simulink model "CLVF"  (R2020a)
settings: Solver=FixedStepAuto  StartTime=0.0  StopTime=tsim  FixedStep=baseRate  RelTol=1e-3  EnableMultiTasking=on
values from neighbouring files (symbols this model uses):
  a = sqrt(sum(aTimesOVec.^2))    [Run_Initializer.m]    (also in a_max_CLVF2D.m = params(4))
  a_max = 0.4/BLACKMass    [Run_Initializer.m]
  a_prime = newParams(2)    [Run_Initializer.m]    (also in a_max_LVF.m = params(2))
  acceptableRadius = 0.05    [Run_Initializer.m]
  b = newParams(3)    [Run_Initializer.m]    (also in a_max_CLVF2D.m = params(3))
  baseRate = 0.05    [Run_Initializer.m]
  BLACKMass = model_param(3)    [Run_Initializer.m]
  d = [0.16;0.542;0]    [Run_Initializer.m]    (also in a_max_LVF.m = [rotStuff(3);rotStuff(4);rotStuff(5)])
  drop_states_BLACK = rC_I0    [Run_Initializer.m]
  drop_states_BLUE = [ xLength/2+0.9; yLength/2+0.5; 0]    [Run_Initializer.m]
  drop_states_RED = rT_I0    [Run_Initializer.m]
  F_thrusters_BLACK = 0.25.*ones(8,1)    [Run_Initializer.m]
  F_thrusters_BLUE = 0.25.*ones(8,1)    [Run_Initializer.m]
  F_thrusters_RED = 0.25.*ones(8,1)    [Run_Initializer.m]
  home_states_BLACK = [ xLength/2+0.4; yLength/2; 0]    [Run_Initializer.m]
  home_states_BLUE = [ xLength/2-0.9; yLength/2+0.5; 0]    [Run_Initializer.m]
  home_states_RED = [ xLength/2-0.4; yLength/2; 0]    [Run_Initializer.m]
  init_states_BLACK = rC_I0    [Run_Initializer.m]
  init_states_BLUE = [ xLength/2+0.9; yLength/2+0.5; 0]    [Run_Initializer.m]
  init_states_RED = rT_I0    [Run_Initializer.m]
  k_v_rel = 2*v_max/a_prime    (= 1)    [Run_Initializer.m]
  ka = newParams(2)    [Run_Initializer.m]    (also in a_max_CLVF2D.m = params(2))
  kc = newParams(1)    [Run_Initializer.m]    (also in a_max_CLVF2D.m = params(1))
  kd = 5.0    (= 5)    [Run_Initializer.m]
  Kd_tb = 0.4    [Run_Initializer.m]
  Kd_tblue = 0.4    [Run_Initializer.m]
  Kd_tr = 0.4    [Run_Initializer.m]
  Kd_xb = 5    [Run_Initializer.m]
  Kd_xblue = 5    [Run_Initializer.m]
  Kd_xr = 5    [Run_Initializer.m]
  Kd_yb = 5    [Run_Initializer.m]
  Kd_yblue = 5    [Run_Initializer.m]
  Kd_yr = 5    [Run_Initializer.m]
  Kp_tb = 0.1    [Run_Initializer.m]
  Kp_tblue = 0.1    [Run_Initializer.m]
  Kp_tr = 0.1    [Run_Initializer.m]
  Kp_xb = 2    [Run_Initializer.m]
  Kp_xblue = 2    [Run_Initializer.m]
  Kp_xr = 2    [Run_Initializer.m]
  Kp_yb = 2    [Run_Initializer.m]
  Kp_yblue = 2    [Run_Initializer.m]
  Kp_yr = 2    [Run_Initializer.m]
  noise_variance_BLACK = 0    [Run_Initializer.m]
  noise_variance_BLUE = 0    [Run_Initializer.m]
  noise_variance_RED = 0    [Run_Initializer.m]
  o_hat_B = aTimesOVec./a    [Run_Initializer.m]
  o_hat_prime = o_prime/sqrt(sum(o_prime.^2))    [Run_Initializer.m]
  Phase0_End = Phase0_Duration    (= 10)    [Run_Initializer.m]
  Phase1_End = Phase0_Duration + Phase1_Duration    (= 15)    [Run_Initializer.m]
  Phase2_End = Phase0_Duration + Phase1_Duration +                                   Phase2_Duration    (= 35)    [Run_Initializer.m]
  Phase3_End = Phase0_Duration + Phase1_Duration +                                   Phase2_Duration + Phase3_Duration    [Run_Initializer.m]
  Phase3_SubPhase1_End = Phase2_End + Phase3_SubPhase1_Duration    (= 40)    [Run_Initializer.m]
  Phase3_SubPhase2_End = Phase2_End + Phase3_SubPhase1_Duration +                                   Phase3_SubPhase2_Duration    (= 45)    [Run_Initializer.m]
  Phase3_SubPhase3_End_BLACK = Phase2_End + Phase3_SubPhase1_Duration +                                   Phase3_SubPhase2_Duration +                                  Phase3_SubPhase3_Duration + Phase3_SubPhase3_and_a_half    (= 51)    [Run_Initializer.m]
  Phase3_SubPhase3_End_RED = Phase2_End + Phase3_SubPhase1_Duration +                                   Phase3_SubPhase2_Duration +                                  Phase3_SubPhase3_Duration    (= 46)    [Run_Initializer.m]
  Phase3_SubPhase4_End = Phase2_End + Phase3_SubPhase1_Duration +                                   Phase3_SubPhase2_Duration +                                  Phase3_SubPhase3_Duration +                                  Phase3_SubPhase4_Duration + Phase3_SubPhase3_and_a_half    [Run_Initializer.m]
  Phase4_End = Phase0_Duration + Phase1_Duration +                                   Phase2_Duration + Phase3_Duration +                                   Phase4_Duration    [Run_Initializer.m]
  Phase5_End = Phase0_Duration + Phase1_Duration +                                   Phase2_Duration + Phase3_Duration +                                   Phase4_Duration + Phase5_Duration    [Run_Initializer.m]
  r_co = r_co_over_a_prime*a_prime    (= 0.16)    [Run_Initializer.m]
  rC_I0 = [0.9*xLength;yLength/2-0.5;pi/2]    [Run_Initializer.m]
  rT_I0 = [yLength/2;yLength/2;possibleStarts(startingRotation)]    [Run_Initializer.m]
  serverRate = 0.1    [Run_Initializer.m]
  sys_BLACK = c2d(sys_BLACK_CONT, baseRate)    [Run_Initializer.m]
  sys_BLACK_ROT = c2d(sys_BLACK_rot_CONT, baseRate)    [Run_Initializer.m]
  sys_RED = c2d(sys_RED_CONT, baseRate)    [Run_Initializer.m]
  sys_RED_ROT = c2d(sys_RED_rot_CONT, baseRate)    [Run_Initializer.m]
  theta_d = 30*d2r    (= 0.523598775598)    [Run_Initializer.m]    (also in a_max_LVF.m = rotStuff(2))
  thruster_dist2CG_BLACK = [83.42;-52.58;55.94;-60.05;54.08;-53.92;77.06;-55.94]    [Run_Initializer.m]
  thruster_dist2CG_BLUE = [83.42;-52.58;55.94;-60.05;54.08;-53.92;77.06;-55.94]    [Run_Initializer.m]
  thruster_dist2CG_RED = [49.92;-78.08;70.46;-63.54;81.08;-50.42;57.44;-75.96]    [Run_Initializer.m]
  w_body = 6.0 * d2r    (= 0.10471975512)    [Run_Initializer.m]
undefined symbols (not defined in the file or in its folder): DiscIntNeverNeededParam, Discrete, Phase3_SubPhase3_End, platformSelection, simMode, Time, WhoAmI
libraries: dspstat3 x18, dspsigops x14, raspberrypiBasiclib x10, embdlinuxlib x8, simulink x8, ctrlSharedLib x4, mspfiltlib x3, dsparch4 x3, dspswit3 x2, MainLibrary x2, sensehatlib x1
(part 5 of 10)

== system CLVF/Phase #4: Return Home/Change BLUE Behavior/Custom Discrete PD (Y-Position) ==
  ey : Inport
  Sum3 : Sum
  kd_yb : Gain  Gain=Kd_yblue
  kp_yb : Gain  Gain=Kp_yblue
  "x_dot -> x1" : Subsystem
  Fy : Outport  VectorParamsAs1DForOutWhenUnconnected=off
  wires:
  kd_yb/1 -> Sum3/1
  Sum3/1 -> Fy/1
  kp_yb/1 -> Sum3/2
  "x_dot -> x1"/1(dy(t)/dt) -> kd_yb/1
  ey/1 -> "x_dot -> x1"/1(y(t)), kp_yb/1

== system CLVF/Phase #4: Return Home/Change BLUE Behavior/Hough Control ==
  Ref : Inport
  Act : Inport  Port=2
  MATLAB Function2 : MATLAB Function  TreatAsAtomicUnit=on
  MATLAB Function3 : MATLAB Function  TreatAsAtomicUnit=on
  MATLAB Function4 : MATLAB Function  TreatAsAtomicUnit=on
  Subtract2 : Sum  Inputs=+-
  Err : Outport  VectorParamsAs1DForOutWhenUnconnected=off
  wires:
  MATLAB Function4/1(e_out) -> Err/1
  MATLAB Function2/1(Oy) -> MATLAB Function4/1(Oy)
  Subtract2/1 -> MATLAB Function4/2(e_in)
  MATLAB Function2/2(Ox) -> Subtract2/1
  Act/1 -> MATLAB Function3/1(z)
  Ref/1 -> MATLAB Function2/1(z)
  MATLAB Function3/1(Ox) -> Subtract2/2

== system CLVF/Phase #4: Return Home/Change RED Behavior/Custom Discrete PD (Attitude) ==
  ez : Inport
  Sum3 : Sum
  kd_tr : Gain  Gain=Kd_tr
  kp_tr : Gain  Gain=Kp_tr
  "x_dot -> x1" : Subsystem
  Tz : Outport  VectorParamsAs1DForOutWhenUnconnected=off
  wires:
  kd_tr/1 -> Sum3/1
  Sum3/1 -> Tz/1
  kp_tr/1 -> Sum3/2
  "x_dot -> x1"/1(dy(t)/dt) -> kd_tr/1
  ez/1 -> "x_dot -> x1"/1(y(t)), kp_tr/1

== system CLVF/Phase #4: Return Home/Change RED Behavior/Custom Discrete PD (X-Position) ==
  ex : Inport
  Sum3 : Sum
  kd_xr : Gain  Gain=Kd_xr
  kp_xr : Gain  Gain=Kp_xr
  "x_dot -> x1" : Subsystem
  Fx : Outport  VectorParamsAs1DForOutWhenUnconnected=off
  wires:
  kd_xr/1 -> Sum3/1
  ex/1 -> "x_dot -> x1"/1(y(t)), kp_xr/1
  kp_xr/1 -> Sum3/2
  "x_dot -> x1"/1(dy(t)/dt) -> kd_xr/1
  Sum3/1 -> Fx/1

== system CLVF/Phase #4: Return Home/Change RED Behavior/Custom Discrete PD (Y-Position) ==
  ey : Inport
  Sum3 : Sum
  kd_yr : Gain  Gain=Kd_yr
  kp_yr : Gain  Gain=Kp_yr
  "x_dot -> x1" : Subsystem
  Fy : Outport  VectorParamsAs1DForOutWhenUnconnected=off
  wires:
  kd_yr/1 -> Sum3/1
  Sum3/1 -> Fy/1
  kp_yr/1 -> Sum3/2
  "x_dot -> x1"/1(dy(t)/dt) -> kd_yr/1
  ey/1 -> "x_dot -> x1"/1(y(t)), kp_yr/1

== system CLVF/Phase #4: Return Home/Change RED Behavior/Hough Control ==
  Ref : Inport
  Act : Inport  Port=2
  MATLAB Function2 : MATLAB Function  TreatAsAtomicUnit=on
  MATLAB Function3 : MATLAB Function  TreatAsAtomicUnit=on
  MATLAB Function4 : MATLAB Function  TreatAsAtomicUnit=on
  Subtract2 : Sum  Inputs=+-
  Err : Outport  VectorParamsAs1DForOutWhenUnconnected=off
  wires:
  MATLAB Function4/1(e_out) -> Err/1
  MATLAB Function2/1(Oy) -> MATLAB Function4/1(Oy)
  Subtract2/1 -> MATLAB Function4/2(e_in)
  MATLAB Function2/2(Ox) -> Subtract2/1
  Act/1 -> MATLAB Function3/1(z)
  Ref/1 -> MATLAB Function2/1(z)
  MATLAB Function3/1(Ox) -> Subtract2/2

== system CLVF/Phase #5: Hold Home/Change BLACK Behavior/Custom Discrete PD (Attitude) ==
  ez : Inport
  Sum3 : Sum
  kd_tb : Gain  Gain=Kd_tb
  kp_tb : Gain  Gain=Kp_tb
  "x_dot -> x1" : Subsystem
  Tz : Outport  VectorParamsAs1DForOutWhenUnconnected=off
  wires:
  kd_tb/1 -> Sum3/1
  Sum3/1 -> Tz/1
  kp_tb/1 -> Sum3/2
  "x_dot -> x1"/1(dy(t)/dt) -> kd_tb/1
  ez/1 -> "x_dot -> x1"/1(y(t)), kp_tb/1

== system CLVF/Phase #5: Hold Home/Change BLACK Behavior/Custom Discrete PD (X-Position) ==
  ex : Inport
  Sum3 : Sum
  kd_xb : Gain  Gain=Kd_xb
  kp_xb : Gain  Gain=Kp_xb
  "x_dot -> x1" : Subsystem
  Fx : Outport  VectorParamsAs1DForOutWhenUnconnected=off
  wires:
  kd_xb/1 -> Sum3/1
  ex/1 -> "x_dot -> x1"/1(y(t)), kp_xb/1
  kp_xb/1 -> Sum3/2
  "x_dot -> x1"/1(dy(t)/dt) -> kd_xb/1
  Sum3/1 -> Fx/1

== system CLVF/Phase #5: Hold Home/Change BLACK Behavior/Custom Discrete PD (Y-Position) ==
  ey : Inport
  Sum3 : Sum
  kd_yb : Gain  Gain=Kd_yb
  kp_yb : Gain  Gain=Kp_yb
  "x_dot -> x1" : Subsystem
  Fy : Outport  VectorParamsAs1DForOutWhenUnconnected=off
  wires:
  kd_yb/1 -> Sum3/1
  Sum3/1 -> Fy/1
  kp_yb/1 -> Sum3/2
  "x_dot -> x1"/1(dy(t)/dt) -> kd_yb/1
  ey/1 -> "x_dot -> x1"/1(y(t)), kp_yb/1

== system CLVF/Phase #5: Hold Home/Change BLACK Behavior/Hough Control ==
  Ref : Inport
  Act : Inport  Port=2
  MATLAB Function2 : MATLAB Function  TreatAsAtomicUnit=on
  MATLAB Function3 : MATLAB Function  TreatAsAtomicUnit=on
  MATLAB Function4 : MATLAB Function  TreatAsAtomicUnit=on
  Subtract2 : Sum  Inputs=+-
  Err : Outport  VectorParamsAs1DForOutWhenUnconnected=off
  wires:
  MATLAB Function4/1(e_out) -> Err/1
  MATLAB Function2/1(Oy) -> MATLAB Function4/1(Oy)
  Subtract2/1 -> MATLAB Function4/2(e_in)
  MATLAB Function2/2(Ox) -> Subtract2/1
  Act/1 -> MATLAB Function3/1(z)
  Ref/1 -> MATLAB Function2/1(z)
  MATLAB Function3/1(Ox) -> Subtract2/2

== system CLVF/Phase #5: Hold Home/Change BLUE Behavior/Custom Discrete PD (Attitude) ==
  ez : Inport
  Sum3 : Sum
  kd_tb : Gain  Gain=Kd_tblue
  kp_tb : Gain  Gain=Kp_tblue
  "x_dot -> x1" : Subsystem
  Tz : Outport  VectorParamsAs1DForOutWhenUnconnected=off
  wires:
  kd_tb/1 -> Sum3/1
  Sum3/1 -> Tz/1
  kp_tb/1 -> Sum3/2
  "x_dot -> x1"/1(dy(t)/dt) -> kd_tb/1
  ez/1 -> "x_dot -> x1"/1(y(t)), kp_tb/1

== system CLVF/Phase #5: Hold Home/Change BLUE Behavior/Custom Discrete PD (X-Position) ==
  ex : Inport
  Sum3 : Sum
  kd_xb : Gain  Gain=Kd_xblue
  kp_xb : Gain  Gain=Kp_xblue
  "x_dot -> x1" : Subsystem
  Fx : Outport  VectorParamsAs1DForOutWhenUnconnected=off
  wires:
  kd_xb/1 -> Sum3/1
  ex/1 -> "x_dot -> x1"/1(y(t)), kp_xb/1
  kp_xb/1 -> Sum3/2
  "x_dot -> x1"/1(dy(t)/dt) -> kd_xb/1
  Sum3/1 -> Fx/1

== system CLVF/Phase #5: Hold Home/Change BLUE Behavior/Custom Discrete PD (Y-Position) ==
  ey : Inport
  Sum3 : Sum
  kd_yb : Gain  Gain=Kd_yblue
  kp_yb : Gain  Gain=Kp_yblue
  "x_dot -> x1" : Subsystem
  Fy : Outport  VectorParamsAs1DForOutWhenUnconnected=off
  wires:
  kd_yb/1 -> Sum3/1
  Sum3/1 -> Fy/1
  kp_yb/1 -> Sum3/2
  "x_dot -> x1"/1(dy(t)/dt) -> kd_yb/1
  ey/1 -> "x_dot -> x1"/1(y(t)), kp_yb/1

== system CLVF/Phase #5: Hold Home/Change BLUE Behavior/Hough Control ==
  Ref : Inport
  Act : Inport  Port=2
  MATLAB Function2 : MATLAB Function  TreatAsAtomicUnit=on
  MATLAB Function3 : MATLAB Function  TreatAsAtomicUnit=on
  MATLAB Function4 : MATLAB Function  TreatAsAtomicUnit=on
  Subtract2 : Sum  Inputs=+-
  Err : Outport  VectorParamsAs1DForOutWhenUnconnected=off
  wires:
  MATLAB Function4/1(e_out) -> Err/1
  MATLAB Function2/1(Oy) -> MATLAB Function4/1(Oy)
  Subtract2/1 -> MATLAB Function4/2(e_in)
  MATLAB Function2/2(Ox) -> Subtract2/1
  Act/1 -> MATLAB Function3/1(z)
  Ref/1 -> MATLAB Function2/1(z)
  MATLAB Function3/1(Ox) -> Subtract2/2

== system CLVF/Phase #5: Hold Home/Change RED Behavior/Custom Discrete PD (Attitude) ==
  ez : Inport
  Sum3 : Sum
  kd_tr : Gain  Gain=Kd_tr
  kp_tr : Gain  Gain=Kp_tr
  "x_dot -> x1" : Subsystem
  Tz : Outport  VectorParamsAs1DForOutWhenUnconnected=off
  wires:
  kd_tr/1 -> Sum3/1
  Sum3/1 -> Tz/1
  kp_tr/1 -> Sum3/2
  "x_dot -> x1"/1(dy(t)/dt) -> kd_tr/1
  ez/1 -> "x_dot -> x1"/1(y(t)), kp_tr/1

== system CLVF/Phase #5: Hold Home/Change RED Behavior/Custom Discrete PD (X-Position) ==
  ex : Inport
  Sum3 : Sum
  kd_xr : Gain  Gain=Kd_xr
  kp_xr : Gain  Gain=Kp_xr
  "x_dot -> x1" : Subsystem
  Fx : Outport  VectorParamsAs1DForOutWhenUnconnected=off
  wires:
  kd_xr/1 -> Sum3/1
  ex/1 -> "x_dot -> x1"/1(y(t)), kp_xr/1
  kp_xr/1 -> Sum3/2
  "x_dot -> x1"/1(dy(t)/dt) -> kd_xr/1
  Sum3/1 -> Fx/1

== system CLVF/Phase #5: Hold Home/Change RED Behavior/Custom Discrete PD (Y-Position) ==
  ey : Inport
  Sum3 : Sum
  kd_yr : Gain  Gain=Kd_yr
  kp_yr : Gain  Gain=Kp_yr
  "x_dot -> x1" : Subsystem
  Fy : Outport  VectorParamsAs1DForOutWhenUnconnected=off
  wires:
  kd_yr/1 -> Sum3/1
  Sum3/1 -> Fy/1
  kp_yr/1 -> Sum3/2
  "x_dot -> x1"/1(dy(t)/dt) -> kd_yr/1
  ey/1 -> "x_dot -> x1"/1(y(t)), kp_yr/1

== system CLVF/Phase #5: Hold Home/Change RED Behavior/Hough Control ==
  Ref : Inport
  Act : Inport  Port=2
  MATLAB Function2 : MATLAB Function  TreatAsAtomicUnit=on
  MATLAB Function3 : MATLAB Function  TreatAsAtomicUnit=on
  MATLAB Function4 : MATLAB Function  TreatAsAtomicUnit=on
  Subtract2 : Sum  Inputs=+-
  Err : Outport  VectorParamsAs1DForOutWhenUnconnected=off
  wires:
  MATLAB Function4/1(e_out) -> Err/1
  MATLAB Function2/1(Oy) -> MATLAB Function4/1(Oy)
  Subtract2/1 -> MATLAB Function4/2(e_in)
  MATLAB Function2/2(Ox) -> Subtract2/1
  Act/1 -> MATLAB Function3/1(z)
  Ref/1 -> MATLAB Function2/1(z)
  MATLAB Function3/1(Ox) -> Subtract2/2

== system CLVF/Simulate Plant Dynamics/x_dot -> x1/Hold this value ==
  In1 : Inport
  Action Port : ActionPort
  Out1 : Outport  VectorParamsAs1DForOutWhenUnconnected=off
  wires:
  In1/1 -> Out1/1

== system CLVF/Simulate Plant Dynamics/x_dot -> x10/Hold this value ==
  In1 : Inport
  Action Port : ActionPort
  Out1 : Outport  VectorParamsAs1DForOutWhenUnconnected=off
  wires:
  In1/1 -> Out1/1

== system CLVF/Simulate Plant Dynamics/x_dot -> x11/Hold this value ==
  In1 : Inport
  Action Port : ActionPort
  Out1 : Outport  VectorParamsAs1DForOutWhenUnconnected=off
  wires:
  In1/1 -> Out1/1

== system CLVF/Simulate Plant Dynamics/x_dot -> x13/Hold this value ==
  In1 : Inport
  Action Port : ActionPort
  Out1 : Outport  VectorParamsAs1DForOutWhenUnconnected=off
  wires:
  In1/1 -> Out1/1

== system CLVF/Simulate Plant Dynamics/x_dot -> x14/Hold this value ==
  In1 : Inport
  Action Port : ActionPort
  Out1 : Outport  VectorParamsAs1DForOutWhenUnconnected=off
  wires:
  In1/1 -> Out1/1

== system CLVF/Simulate Plant Dynamics/x_dot -> x16/Hold this value ==
  In1 : Inport
  Action Port : ActionPort
  Out1 : Outport  VectorParamsAs1DForOutWhenUnconnected=off
  wires:
  In1/1 -> Out1/1

== system CLVF/Simulate Plant Dynamics/x_dot -> x17/Hold this value ==
  In1 : Inport
  Action Port : ActionPort
  Out1 : Outport  VectorParamsAs1DForOutWhenUnconnected=off
  wires:
  In1/1 -> Out1/1

== system CLVF/Simulate Plant Dynamics/x_dot -> x2/Hold this value ==
  In1 : Inport
  Action Port : ActionPort
  Out1 : Outport  VectorParamsAs1DForOutWhenUnconnected=off
  wires:
  In1/1 -> Out1/1

== system CLVF/Simulate Plant Dynamics/x_dot -> x3/Hold this value ==
  In1 : Inport
  Action Port : ActionPort
  Out1 : Outport  VectorParamsAs1DForOutWhenUnconnected=off
  wires:
  In1/1 -> Out1/1

== system CLVF/Simulate Plant Dynamics/x_dot -> x4/Hold this value ==
  In1 : Inport
  Action Port : ActionPort
  Out1 : Outport  VectorParamsAs1DForOutWhenUnconnected=off
  wires:
  In1/1 -> Out1/1

== system CLVF/Simulate Plant Dynamics/x_dot -> x5/Hold this value ==
  In1 : Inport
  Action Port : ActionPort
  Out1 : Outport  VectorParamsAs1DForOutWhenUnconnected=off
  wires:
  In1/1 -> Out1/1

== system CLVF/Simulate Plant Dynamics/x_dot -> x6/Hold this value ==
  In1 : Inport
  Action Port : ActionPort
  Out1 : Outport  VectorParamsAs1DForOutWhenUnconnected=off
  wires:
  In1/1 -> Out1/1

== system CLVF/Simulate Plant Dynamics/x_dot -> x7/Hold this value ==
  In1 : Inport
  Action Port : ActionPort
  Out1 : Outport  VectorParamsAs1DForOutWhenUnconnected=off
  wires:
  In1/1 -> Out1/1

== system CLVF/Simulate Plant Dynamics/x_dot -> x8/Hold this value ==
  In1 : Inport
  Action Port : ActionPort
  Out1 : Outport  VectorParamsAs1DForOutWhenUnconnected=off
  wires:
  In1/1 -> Out1/1

== system CLVF/Simulate Plant Dynamics/x_dot -> x9/Hold this value ==
  In1 : Inport
  Action Port : ActionPort
  Out1 : Outport  VectorParamsAs1DForOutWhenUnconnected=off
  wires:
  In1/1 -> Out1/1

== system CLVF/From Force//Torque to PWM Signal/Change BLACK Behavior/Calculate Thruster ON//OFF/Rotate Forces to Inertial ==
  "F_b " : Inport
  Rz : Inport  Port=2
  Create Rotation Matrix : MATLAB Function  TreatAsAtomicUnit=on
  Rotate F_b to F_I : Product  Multiplication=Matrix(*)
  F_I : Outport  VectorParamsAs1DForOutWhenUnconnected=off
  wires:
  "F_b "/1 -> Rotate F_b to F_I/2
  Rotate F_b to F_I/1 -> F_I/1
  Create Rotation Matrix/1(C_Ib) -> Rotate F_b to F_I/1
  Rz/1 -> Create Rotation Matrix/1(Rz)

== system CLVF/From Force//Torque to PWM Signal/Change BLACK Behavior/Calculate Thruster ON//OFF/pseudo-inverse ==
  H : Inport
  Product : Product  Multiplication=Matrix(*)
  Product1 : Product  Inputs=/  Multiplication=Matrix(*)
  Product2 : Product  Multiplication=Matrix(*)
  transpose : PermuteDimensions
  invH : Outport  VectorParamsAs1DForOutWhenUnconnected=off
  wires:
  Product2/1 -> invH/1
  transpose/1 -> Product/2, Product2/1
  Product/1 -> Product1/1
  H/1 -> Product/1, transpose/1
  Product1/1 -> Product2/2

== system CLVF/From Force//Torque to PWM Signal/Change BLUE Behavior/Calculate Thruster ON//OFF/Rotate Forces to Inertial ==
  "F_b " : Inport
  Rz : Inport  Port=2
  Create Rotation Matrix : MATLAB Function  TreatAsAtomicUnit=on
  Rotate F_b to F_I : Product  Multiplication=Matrix(*)
  F_I : Outport  VectorParamsAs1DForOutWhenUnconnected=off
  wires:
  "F_b "/1 -> Rotate F_b to F_I/2
  Rotate F_b to F_I/1 -> F_I/1
  Create Rotation Matrix/1(C_Ib) -> Rotate F_b to F_I/1
  Rz/1 -> Create Rotation Matrix/1(Rz)

== system CLVF/From Force//Torque to PWM Signal/Change BLUE Behavior/Calculate Thruster ON//OFF/pseudo-inverse ==
  H : Inport
  Product : Product  Multiplication=Matrix(*)
  Product1 : Product  Inputs=/  Multiplication=Matrix(*)
  Product2 : Product  Multiplication=Matrix(*)
  transpose : PermuteDimensions
  invH : Outport  VectorParamsAs1DForOutWhenUnconnected=off
  wires:
  Product2/1 -> invH/1
  transpose/1 -> Product/2, Product2/1
  Product/1 -> Product1/1
  H/1 -> Product/1, transpose/1
  Product1/1 -> Product2/2

== system CLVF/From Force//Torque to PWM Signal/Change RED Behavior/Calculate Thruster ON//OFF/Rotate Forces to Inertial ==
  "F_b " : Inport
  Rz : Inport  Port=2
  Create Rotation Matrix : MATLAB Function  TreatAsAtomicUnit=on
  Rotate F_b to F_I : Product  Multiplication=Matrix(*)
  F_I : Outport  VectorParamsAs1DForOutWhenUnconnected=off
  wires:
  "F_b "/1 -> Rotate F_b to F_I/2
  Rotate F_b to F_I/1 -> F_I/1
  Create Rotation Matrix/1(C_Ib) -> Rotate F_b to F_I/1
  Rz/1 -> Create Rotation Matrix/1(Rz)

== system CLVF/From Force//Torque to PWM Signal/Change RED Behavior/Calculate Thruster ON//OFF/pseudo-inverse ==
  H : Inport
  Product : Product  Multiplication=Matrix(*)
  Product1 : Product  Inputs=/  Multiplication=Matrix(*)
  Product2 : Product  Multiplication=Matrix(*)
  transpose : PermuteDimensions
  invH : Outport  VectorParamsAs1DForOutWhenUnconnected=off
  wires:
  Product2/1 -> invH/1
  transpose/1 -> Product/2, Product2/1
  Product/1 -> Product1/1
  H/1 -> Product/1, transpose/1
  Product1/1 -> Product2/2

== system CLVF/From Torque, Command RW/Change RED Behavior/Wheel RPM to PWM/Convert Wheel Rate to Motor Rate ==
  Wheel RPM : Inport
  Divide : Product  Inputs=**
  Gearbox Ratio : Constant  Value=3375/64
  Motor RPM : Outport  VectorParamsAs1DForOutWhenUnconnected=off
  wires:
  Gearbox Ratio/1 -> Divide/2
  Divide/1 -> Motor RPM/1
  Wheel RPM/1 -> Divide/1

== system CLVF/From Torque, Command RW/Change RED Behavior/Wheel RPM to PWM/Delay Bank ==
  Status : Inport
  Delay1 : Delay  DelayLength=1  InitialCondition=0
  Delay2 : Delay  InitialCondition=0
  Delay3 : Delay  DelayLength=4  InitialCondition=0
  Delay4 : Delay  DelayLength=5  InitialCondition=0
  Delay5 : Delay  DelayLength=3  InitialCondition=0
  Mostly zeros? : MinMax  Inputs=6
  StatusVector : Outport  VectorParamsAs1DForOutWhenUnconnected=off
  wires:
  Delay3/1 -> Mostly zeros?/5
  Status/1 -> Delay4/1, Delay3/1, Delay5/1, Delay2/1, Delay1/1, Mostly zeros?/1
  Delay2/1 -> Mostly zeros?/3
  Delay4/1 -> Mostly zeros?/6
  Delay5/1 -> Mostly zeros?/4
  Mostly zeros?/1 -> StatusVector/1
  Delay1/1 -> Mostly zeros?/2

== system CLVF/From Torque, Command RW/Change RED Behavior/Wheel RPM to PWM/Obtain RW Status ==
  GPIO Read1 : embdlinuxlib/GPIO Read  board=Pi 3 Model B  gpio=24  internalResistor=Off  sampleTime=0.1  direction=Input  blockPlatform=Raspberry Pi
      settings: SourceProductBaseCode=SC_BEAGLEBONE_BLUE,RASPPI
  RW_Status : Outport  VectorParamsAs1DForOutWhenUnconnected=off
  wires:
  GPIO Read1/1 -> RW_Status/1

== system CLVF/From Torque, Command RW/Change RED Behavior/Wheel RPM to PWM/Send Direction to Motor Controller ==
  WheelDir : Inport
  GPIO Write : embdlinuxlib/GPIO Write  board=Pi 3 Model B  gpio=21  direction=Output  blockPlatform=Raspberry Pi
      settings: SourceProductBaseCode=SC_BEAGLEBONE_BLUE,RASPPI
  wires:
  WheelDir/1 -> GPIO Write/1

== system CLVF/From Torque, Command RW/Change RED Behavior/Wheel RPM to PWM/Send PWM to Motor Controller ==
  MotorPWM : Inport
  PWM1 : raspberrypiBasiclib/PWM  board=Pi 3 Model B  Pin_=18  Frequency=10  blockPlatform=Raspberry Pi
      settings: SourceProductBaseCode=RASPPI
  wires:
  MotorPWM/1 -> PWM1/1

== system CLVF/From Torque, Command RW/Change RED Behavior/Wheel RPM to PWM/Turn on Motor ==
  EnableSig : Inport
  GPIO Write1 : embdlinuxlib/GPIO Write  board=Pi 3 Model B  gpio=25  direction=Output  blockPlatform=Raspberry Pi
      settings: SourceProductBaseCode=SC_BEAGLEBONE_BLUE,RASPPI
  wires:
  EnableSig/1 -> GPIO Write1/1

== system CLVF/Grab PhaseSpace Data via UDP/Use Hardware to Obtain States/Using RED+BLACK, or RED+BLACK+ARM/Is this a simulation? ==
  Constant : Constant  Value=simMode  SampleTime=-1
  isSim : Outport  VectorParamsAs1DForOutWhenUnconnected=off
  wires:
  Constant/1 -> isSim/1

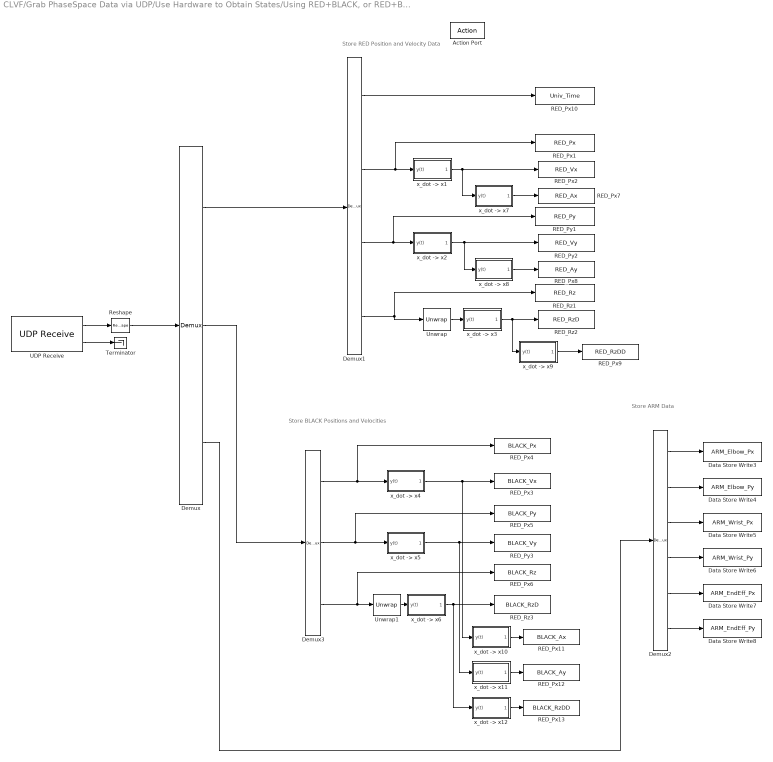
== system CLVF/Grab PhaseSpace Data via UDP/Use Hardware to Obtain States/Using RED+BLACK, or RED+BLACK+ARM/Obtain BLACK States ==
  note: Store ARM Data
  note: Store RED Position and Velocity Data
  note: Store BLACK Positions and Velocities
  Action Port : ActionPort
  Data Store Write3 : DataStoreWrite  DataStoreName=ARM_Elbow_Px
  Data Store Write4 : DataStoreWrite  DataStoreName=ARM_Elbow_Py
  Data Store Write5 : DataStoreWrite  DataStoreName=ARM_Wrist_Px
  Data Store Write6 : DataStoreWrite  DataStoreName=ARM_Wrist_Py
  Data Store Write7 : DataStoreWrite  DataStoreName=ARM_EndEff_Px
  Data Store Write8 : DataStoreWrite  DataStoreName=ARM_EndEff_Py
  Demux : Demux  Outputs=[4,3,6]
  Demux1 : Demux
  Demux2 : Demux  Outputs=6
  Demux3 : Demux  Outputs=3
  RED_Px1 : DataStoreWrite  DataStoreName=RED_Px
  RED_Px10 : DataStoreWrite  DataStoreName=Univ_Time
  RED_Px11 : DataStoreWrite  DataStoreName=BLACK_Ax
  RED_Px12 : DataStoreWrite  DataStoreName=BLACK_Ay
  RED_Px13 : DataStoreWrite  DataStoreName=BLACK_RzDD
  RED_Px2 : DataStoreWrite  DataStoreName=RED_Vx
  RED_Px3 : DataStoreWrite  DataStoreName=BLACK_Vx
  RED_Px4 : DataStoreWrite  DataStoreName=BLACK_Px
  RED_Px5 : DataStoreWrite  DataStoreName=BLACK_Py
  RED_Px6 : DataStoreWrite  DataStoreName=BLACK_Rz
  RED_Px7 : DataStoreWrite  DataStoreName=RED_Ax
  RED_Px8 : DataStoreWrite  DataStoreName=RED_Ay
  RED_Px9 : DataStoreWrite  DataStoreName=RED_RzDD
  RED_Py1 : DataStoreWrite  DataStoreName=RED_Py
  RED_Py2 : DataStoreWrite  DataStoreName=RED_Vy
  RED_Py3 : DataStoreWrite  DataStoreName=BLACK_Vy
  RED_Rz1 : DataStoreWrite  DataStoreName=RED_Rz
  RED_Rz2 : DataStoreWrite  DataStoreName=RED_RzD
  RED_Rz3 : DataStoreWrite  DataStoreName=BLACK_RzD
  Reshape : Reshape  OutputDimensionality=Customize  OutputDimensions=[13,1]
  Terminator : Terminator
  UDP Receive : embdlinuxlib/UDP Receive  localURL='0.0.0.0'  localPort=25000  remoteURL='0.0.0.0'  remotePort=-1  recvBufferSize=8192  signalDatatype=double  dims=13  isVarSize=off  showBlockingTime=off  blockingTime=0  sampletime=-1  blockPlatform=Raspberry Pi
      settings: SourceProductBaseCode=SC_BEAGLEBONE_BLUE,RASPPI
  Unwrap : dspsigops/Unwrap  tol=pi  InputProcessing=Columns as channels (frame based)  running=off
  Unwrap1 : dspsigops/Unwrap  tol=pi  InputProcessing=Columns as channels (frame based)  running=off
  "x_dot -> x1" : Subsystem
  "x_dot -> x10" : Subsystem
  "x_dot -> x11" : Subsystem
  "x_dot -> x12" : Subsystem
  "x_dot -> x2" : Subsystem
  "x_dot -> x3" : Subsystem
  "x_dot -> x4" : Subsystem
  "x_dot -> x5" : Subsystem
  "x_dot -> x6" : Subsystem
  "x_dot -> x7" : Subsystem
  "x_dot -> x8" : Subsystem
  "x_dot -> x9" : Subsystem
  wires:
  UDP Receive/1 -> Reshape/1
  UDP Receive/2 -> Terminator/1
  "x_dot -> x8"/1(dy(t)/dt) -> RED_Px8/1
  Demux2/2 -> Data Store Write4/1
  Reshape/1 -> Demux/1
  Demux1/4 -> Unwrap/1, RED_Rz1/1
  Demux1/1 -> RED_Px10/1
  Unwrap/1 -> "x_dot -> x3"/1(y(t))
  "x_dot -> x7"/1(dy(t)/dt) -> RED_Px7/1
  Demux/2 -> Demux3/1
  "x_dot -> x9"/1(dy(t)/dt) -> RED_Px9/1
  Demux/1 -> Demux1/1
  Demux/3 -> Demux2/1
  "x_dot -> x3"/1(dy(t)/dt) -> "x_dot -> x9"/1(y(t)), RED_Rz2/1
  "x_dot -> x1"/1(dy(t)/dt) -> "x_dot -> x7"/1(y(t)), RED_Px2/1
  Demux1/2 -> "x_dot -> x1"/1(y(t)), RED_Px1/1
  Demux2/4 -> Data Store Write6/1
  Demux2/6 -> Data Store Write8/1
  "x_dot -> x2"/1(dy(t)/dt) -> "x_dot -> x8"/1(y(t)), RED_Py2/1
  Demux2/3 -> Data Store Write5/1
  Demux1/3 -> "x_dot -> x2"/1(y(t)), RED_Py1/1
  Demux2/1 -> Data Store Write3/1
  Demux2/5 -> Data Store Write7/1
  "x_dot -> x11"/1(dy(t)/dt) -> RED_Px12/1
  Demux3/2 -> "x_dot -> x5"/1(y(t)), RED_Px5/1
  Demux3/3 -> Unwrap1/1, RED_Px6/1
  "x_dot -> x5"/1(dy(t)/dt) -> RED_Py3/1, "x_dot -> x11"/1(y(t))
  "x_dot -> x4"/1(dy(t)/dt) -> "x_dot -> x10"/1(y(t)), RED_Px3/1
  "x_dot -> x6"/1(dy(t)/dt) -> RED_Rz3/1, "x_dot -> x12"/1(y(t))
  Unwrap1/1 -> "x_dot -> x6"/1(y(t))
  "x_dot -> x12"/1(dy(t)/dt) -> RED_Px13/1
  Demux3/1 -> "x_dot -> x4"/1(y(t)), RED_Px4/1
  "x_dot -> x10"/1(dy(t)/dt) -> RED_Px11/1

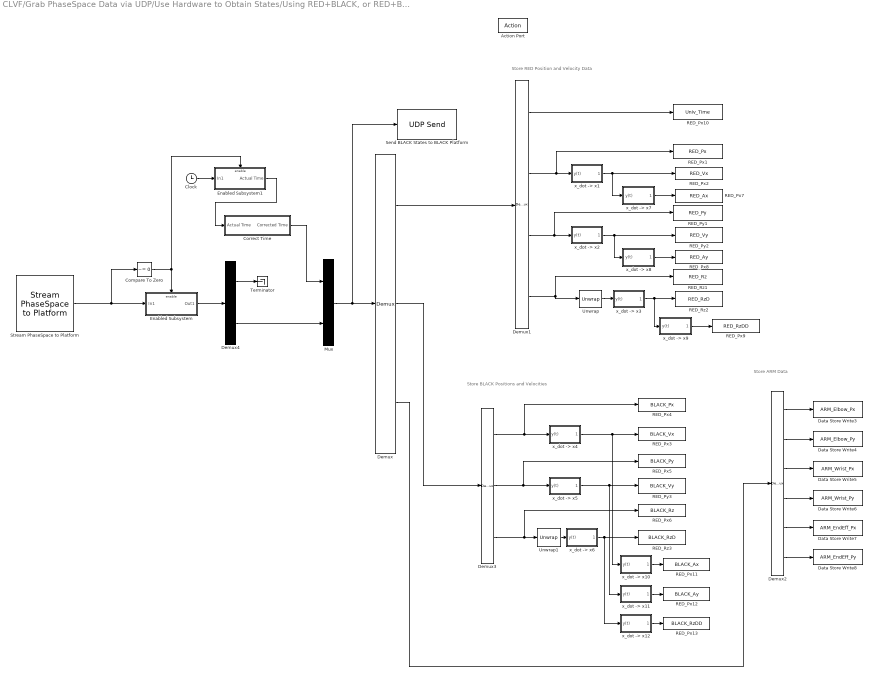
== system CLVF/Grab PhaseSpace Data via UDP/Use Hardware to Obtain States/Using RED+BLACK, or RED+BLACK+ARM/Obtain RED States ==
  note: Store ARM Data
  note: Store RED Position and Velocity Data
  note: Store BLACK Positions and Velocities
  Action Port : ActionPort
  Clock : Clock
  Compare To Zero : simulink/Logic and Bit Operations/Compare To Zero  relop=~=  OutDataTypeStr=boolean
  Correct Time : Subsystem
  Data Store Write3 : DataStoreWrite  DataStoreName=ARM_Elbow_Px
  Data Store Write4 : DataStoreWrite  DataStoreName=ARM_Elbow_Py
  Data Store Write5 : DataStoreWrite  DataStoreName=ARM_Wrist_Px
  Data Store Write6 : DataStoreWrite  DataStoreName=ARM_Wrist_Py
  Data Store Write7 : DataStoreWrite  DataStoreName=ARM_EndEff_Px
  Data Store Write8 : DataStoreWrite  DataStoreName=ARM_EndEff_Py
  Demux : Demux  Outputs=[4,3,6]
  Demux1 : Demux
  Demux2 : Demux  Outputs=6
  Demux3 : Demux  Outputs=3
  Demux4 : Demux  Outputs=[1,12]
  Enabled Subsystem : Subsystem  TreatAsAtomicUnit=on
  Enabled Subsystem1 : Subsystem  TreatAsAtomicUnit=on
  Mux : Mux  Inputs=2
  RED_Px1 : DataStoreWrite  DataStoreName=RED_Px
  RED_Px10 : DataStoreWrite  DataStoreName=Univ_Time
  RED_Px11 : DataStoreWrite  DataStoreName=BLACK_Ax
  RED_Px12 : DataStoreWrite  DataStoreName=BLACK_Ay
  RED_Px13 : DataStoreWrite  DataStoreName=BLACK_RzDD
  RED_Px2 : DataStoreWrite  DataStoreName=RED_Vx
  RED_Px3 : DataStoreWrite  DataStoreName=BLACK_Vx
  RED_Px4 : DataStoreWrite  DataStoreName=BLACK_Px
  RED_Px5 : DataStoreWrite  DataStoreName=BLACK_Py
  RED_Px6 : DataStoreWrite  DataStoreName=BLACK_Rz
  RED_Px7 : DataStoreWrite  DataStoreName=RED_Ax
  RED_Px8 : DataStoreWrite  DataStoreName=RED_Ay
  RED_Px9 : DataStoreWrite  DataStoreName=RED_RzDD
  RED_Py1 : DataStoreWrite  DataStoreName=RED_Py
  RED_Py2 : DataStoreWrite  DataStoreName=RED_Vy
  RED_Py3 : DataStoreWrite  DataStoreName=BLACK_Vy
  RED_Rz1 : DataStoreWrite  DataStoreName=RED_Rz
  RED_Rz2 : DataStoreWrite  DataStoreName=RED_RzD
  RED_Rz3 : DataStoreWrite  DataStoreName=BLACK_RzD
  Send BLACK States to BLACK Platform : embdlinuxlib/UDP Send  remoteURL='192.168.0.101'  remotePort=25000  localURL='255.255.255.255'  localPortSource=Automatically determine  localPort=-1  sampletime=-1  blockPlatform=Raspberry Pi  separateLengthPort=0
      settings: SourceProductBaseCode=SC_BEAGLEBONE_BLUE,RASPPI
  Stream PhaseSpace to Platform : MainLibrary/PhaseSpace Functions/Stream PhaseSpace to Platform  platformSelection=platformSelection  PS_SampleRate=1/serverRate
      settings: SourceProductName=SPOT Custom Library
  Terminator : Terminator
  Unwrap : dspsigops/Unwrap  tol=pi  InputProcessing=Columns as channels (frame based)  running=off
  Unwrap1 : dspsigops/Unwrap  tol=pi  InputProcessing=Columns as channels (frame based)  running=off
  "x_dot -> x1" : Subsystem
  "x_dot -> x10" : Subsystem
  "x_dot -> x11" : Subsystem
  "x_dot -> x12" : Subsystem
  "x_dot -> x2" : Subsystem
  "x_dot -> x3" : Subsystem
  "x_dot -> x4" : Subsystem
  "x_dot -> x5" : Subsystem
  "x_dot -> x6" : Subsystem
  "x_dot -> x7" : Subsystem
  "x_dot -> x8" : Subsystem
  "x_dot -> x9" : Subsystem
  wires:
  "x_dot -> x8"/1(dy(t)/dt) -> RED_Px8/1
  Demux2/2 -> Data Store Write4/1
  Demux1/4 -> Unwrap/1, RED_Rz1/1
  Demux1/1 -> RED_Px10/1
  Unwrap/1 -> "x_dot -> x3"/1(y(t))
  "x_dot -> x7"/1(dy(t)/dt) -> RED_Px7/1
  Demux/2 -> Demux3/1
  "x_dot -> x9"/1(dy(t)/dt) -> RED_Px9/1
  Demux/1 -> Demux1/1
  Demux/3 -> Demux2/1
  "x_dot -> x3"/1(dy(t)/dt) -> "x_dot -> x9"/1(y(t)), RED_Rz2/1
  "x_dot -> x1"/1(dy(t)/dt) -> "x_dot -> x7"/1(y(t)), RED_Px2/1
  Demux1/2 -> "x_dot -> x1"/1(y(t)), RED_Px1/1
  Demux2/4 -> Data Store Write6/1
  Demux2/6 -> Data Store Write8/1
  "x_dot -> x2"/1(dy(t)/dt) -> "x_dot -> x8"/1(y(t)), RED_Py2/1
  Demux2/3 -> Data Store Write5/1
  Demux1/3 -> "x_dot -> x2"/1(y(t)), RED_Py1/1
  Demux2/1 -> Data Store Write3/1
  Demux2/5 -> Data Store Write7/1
  "x_dot -> x11"/1(dy(t)/dt) -> RED_Px12/1
  Demux3/2 -> "x_dot -> x5"/1(y(t)), RED_Px5/1
  Demux3/3 -> Unwrap1/1, RED_Px6/1
  "x_dot -> x5"/1(dy(t)/dt) -> RED_Py3/1, "x_dot -> x11"/1(y(t))
  "x_dot -> x4"/1(dy(t)/dt) -> "x_dot -> x10"/1(y(t)), RED_Px3/1
  "x_dot -> x6"/1(dy(t)/dt) -> RED_Rz3/1, "x_dot -> x12"/1(y(t))
  Unwrap1/1 -> "x_dot -> x6"/1(y(t))
  "x_dot -> x12"/1(dy(t)/dt) -> RED_Px13/1
  Demux3/1 -> "x_dot -> x4"/1(y(t)), RED_Px4/1
  "x_dot -> x10"/1(dy(t)/dt) -> RED_Px11/1
  Enabled Subsystem1/1(Actual Time) -> Correct Time/1(Actual Time)
  Demux4/1 -> Terminator/1
  Correct Time/1(Corrected Time) -> Mux/1
  Clock/1 -> Enabled Subsystem1/1(In1)
  Stream PhaseSpace to Platform/1 -> Enabled Subsystem/1(In1), Compare To Zero/1
  Compare To Zero/1 -> Enabled Subsystem1/Enable, Enabled Subsystem/Enable
  Demux4/2 -> Mux/2
  Enabled Subsystem/1(Out1) -> Demux4/1
  Mux/1 -> Send BLACK States to BLACK Platform/1, Demux/1

== system CLVF/Grab PhaseSpace Data via UDP/Use Hardware to Obtain States/Using RED, BLACK, BLUE, or RED + ARM/Correct Time ==
  Actual Time : Inport
  Edge Detector : dspswit3/Edge Detector  InputProcessing=Columns as channels (frame based)
      settings: SourceProductBaseCode=DS
  Enabled Subsystem : Subsystem  TreatAsAtomicUnit=on
  Subtract : Sum  Inputs=+-
  Corrected Time : Outport  VectorParamsAs1DForOutWhenUnconnected=off
  wires:
  Subtract/1 -> Corrected Time/1
  Edge Detector/1 -> Enabled Subsystem/Enable
  Actual Time/1 -> Subtract/1, Enabled Subsystem/1(In1), Edge Detector/1
  Enabled Subsystem/1(Out1) -> Subtract/2

== system CLVF/Grab PhaseSpace Data via UDP/Use Hardware to Obtain States/Using RED, BLACK, BLUE, or RED + ARM/Enabled Subsystem ==
  In1 : Inport
  Enable : EnablePort
  Out1 : Outport  VectorParamsAs1DForOutWhenUnconnected=off
  wires:
  In1/1 -> Out1/1

== system CLVF/Grab PhaseSpace Data via UDP/Use Hardware to Obtain States/Using RED, BLACK, BLUE, or RED + ARM/Enabled Subsystem1 ==
  In1 : Inport
  Enable : EnablePort
  Actual Time : Outport  VectorParamsAs1DForOutWhenUnconnected=off
  wires:
  In1/1 -> Actual Time/1

== system CLVF/Grab PhaseSpace Data via UDP/Use Hardware to Obtain States/Using RED, BLACK, BLUE, or RED + ARM/x_dot -> x1 ==
  note: dy/dt ~= (y2-y1)/deltaT
  y(t) : Inport
  Delay1 : Delay  DelayLength=1  InitialConditionSource=Input port
      settings: InputPortMap=u0,p4
  Hold this value : Subsystem  TreatAsAtomicUnit=on
  Sum6 : Sum  Inputs=-+|
  divide by delta T : Gain  Gain=1/serverRate
  "if we went through a \"step\"" : If  IfExpression=u1 ~= 0  ShowElse=off
  dy(t)/dt : Outport  VectorParamsAs1DForOutWhenUnconnected=off
  wires:
  divide by delta T/1 -> dy(t)/dt/1
  Delay1/1 -> Sum6/1
  "if we went through a \"step\""/1 -> Hold this value/Action
  Hold this value/1(Out1) -> divide by delta T/1
  Sum6/1 -> "if we went through a \"step\""/1, Hold this value/1(In1)
  y(t)/1 -> Sum6/2, Delay1/2, Delay1/1

== system CLVF/Grab PhaseSpace Data via UDP/Use Hardware to Obtain States/Using RED, BLACK, BLUE, or RED + ARM/x_dot -> x10 ==
  note: dy/dt ~= (y2-y1)/deltaT
  y(t) : Inport
  Delay1 : Delay  DelayLength=1  InitialConditionSource=Input port
      settings: InputPortMap=u0,p4
  Hold this value : Subsystem  TreatAsAtomicUnit=on
  Sum6 : Sum  Inputs=-+|
  divide by delta T : Gain  Gain=1/serverRate
  "if we went through a \"step\"" : If  IfExpression=u1 ~= 0  ShowElse=off
  dy(t)/dt : Outport  VectorParamsAs1DForOutWhenUnconnected=off
  wires:
  divide by delta T/1 -> dy(t)/dt/1
  Delay1/1 -> Sum6/1
  "if we went through a \"step\""/1 -> Hold this value/Action
  Hold this value/1(Out1) -> divide by delta T/1
  Sum6/1 -> "if we went through a \"step\""/1, Hold this value/1(In1)
  y(t)/1 -> Sum6/2, Delay1/2, Delay1/1

== system CLVF/Grab PhaseSpace Data via UDP/Use Hardware to Obtain States/Using RED, BLACK, BLUE, or RED + ARM/x_dot -> x11 ==
  note: dy/dt ~= (y2-y1)/deltaT
  y(t) : Inport
  Delay1 : Delay  DelayLength=1  InitialConditionSource=Input port
      settings: InputPortMap=u0,p4
  Hold this value : Subsystem  TreatAsAtomicUnit=on
  Sum6 : Sum  Inputs=-+|
  divide by delta T : Gain  Gain=1/serverRate
  "if we went through a \"step\"" : If  IfExpression=u1 ~= 0  ShowElse=off
  dy(t)/dt : Outport  VectorParamsAs1DForOutWhenUnconnected=off
  wires:
  divide by delta T/1 -> dy(t)/dt/1
  Delay1/1 -> Sum6/1
  "if we went through a \"step\""/1 -> Hold this value/Action
  Hold this value/1(Out1) -> divide by delta T/1
  Sum6/1 -> "if we went through a \"step\""/1, Hold this value/1(In1)
  y(t)/1 -> Sum6/2, Delay1/2, Delay1/1

== system CLVF/Grab PhaseSpace Data via UDP/Use Hardware to Obtain States/Using RED, BLACK, BLUE, or RED + ARM/x_dot -> x12 ==
  note: dy/dt ~= (y2-y1)/deltaT
  y(t) : Inport
  Delay1 : Delay  DelayLength=1  InitialConditionSource=Input port
      settings: InputPortMap=u0,p4
  Hold this value : Subsystem  TreatAsAtomicUnit=on
  Sum6 : Sum  Inputs=-+|
  divide by delta T : Gain  Gain=1/serverRate
  "if we went through a \"step\"" : If  IfExpression=u1 ~= 0  ShowElse=off
  dy(t)/dt : Outport  VectorParamsAs1DForOutWhenUnconnected=off
  wires:
  divide by delta T/1 -> dy(t)/dt/1
  Delay1/1 -> Sum6/1
  "if we went through a \"step\""/1 -> Hold this value/Action
  Hold this value/1(Out1) -> divide by delta T/1
  Sum6/1 -> "if we went through a \"step\""/1, Hold this value/1(In1)
  y(t)/1 -> Sum6/2, Delay1/2, Delay1/1

== system CLVF/Grab PhaseSpace Data via UDP/Use Hardware to Obtain States/Using RED, BLACK, BLUE, or RED + ARM/x_dot -> x2 ==
  note: dy/dt ~= (y2-y1)/deltaT
  y(t) : Inport
  Delay1 : Delay  DelayLength=1  InitialConditionSource=Input port
      settings: InputPortMap=u0,p4
  Hold this value : Subsystem  TreatAsAtomicUnit=on
  Sum6 : Sum  Inputs=-+|
  divide by delta T : Gain  Gain=1/serverRate
  "if we went through a \"step\"" : If  IfExpression=u1 ~= 0  ShowElse=off
  dy(t)/dt : Outport  VectorParamsAs1DForOutWhenUnconnected=off
  wires:
  divide by delta T/1 -> dy(t)/dt/1
  Delay1/1 -> Sum6/1
  "if we went through a \"step\""/1 -> Hold this value/Action
  Hold this value/1(Out1) -> divide by delta T/1
  Sum6/1 -> "if we went through a \"step\""/1, Hold this value/1(In1)
  y(t)/1 -> Sum6/2, Delay1/2, Delay1/1

== system CLVF/Grab PhaseSpace Data via UDP/Use Hardware to Obtain States/Using RED, BLACK, BLUE, or RED + ARM/x_dot -> x3 ==
  note: dy/dt ~= (y2-y1)/deltaT
  y(t) : Inport
  Delay1 : Delay  DelayLength=1  InitialConditionSource=Input port
      settings: InputPortMap=u0,p4
  Hold this value : Subsystem  TreatAsAtomicUnit=on
  Sum6 : Sum  Inputs=-+|
  divide by delta T : Gain  Gain=1/serverRate
  "if we went through a \"step\"" : If  IfExpression=u1 ~= 0  ShowElse=off
  dy(t)/dt : Outport  VectorParamsAs1DForOutWhenUnconnected=off
  wires:
  divide by delta T/1 -> dy(t)/dt/1
  Delay1/1 -> Sum6/1
  "if we went through a \"step\""/1 -> Hold this value/Action
  Hold this value/1(Out1) -> divide by delta T/1
  Sum6/1 -> "if we went through a \"step\""/1, Hold this value/1(In1)
  y(t)/1 -> Sum6/2, Delay1/2, Delay1/1

== system CLVF/Grab PhaseSpace Data via UDP/Use Hardware to Obtain States/Using RED, BLACK, BLUE, or RED + ARM/x_dot -> x4 ==
  note: dy/dt ~= (y2-y1)/deltaT
  y(t) : Inport
  Delay1 : Delay  DelayLength=1  InitialConditionSource=Input port
      settings: InputPortMap=u0,p4
  Hold this value : Subsystem  TreatAsAtomicUnit=on
  Sum6 : Sum  Inputs=-+|
  divide by delta T : Gain  Gain=1/serverRate
  "if we went through a \"step\"" : If  IfExpression=u1 ~= 0  ShowElse=off
  dy(t)/dt : Outport  VectorParamsAs1DForOutWhenUnconnected=off
  wires:
  divide by delta T/1 -> dy(t)/dt/1
  Delay1/1 -> Sum6/1
  "if we went through a \"step\""/1 -> Hold this value/Action
  Hold this value/1(Out1) -> divide by delta T/1
  Sum6/1 -> "if we went through a \"step\""/1, Hold this value/1(In1)
  y(t)/1 -> Sum6/2, Delay1/2, Delay1/1

== system CLVF/Grab PhaseSpace Data via UDP/Use Hardware to Obtain States/Using RED, BLACK, BLUE, or RED + ARM/x_dot -> x5 ==
  note: dy/dt ~= (y2-y1)/deltaT
  y(t) : Inport
  Delay1 : Delay  DelayLength=1  InitialConditionSource=Input port
      settings: InputPortMap=u0,p4
  Hold this value : Subsystem  TreatAsAtomicUnit=on
  Sum6 : Sum  Inputs=-+|
  divide by delta T : Gain  Gain=1/serverRate
  "if we went through a \"step\"" : If  IfExpression=u1 ~= 0  ShowElse=off
  dy(t)/dt : Outport  VectorParamsAs1DForOutWhenUnconnected=off
  wires:
  divide by delta T/1 -> dy(t)/dt/1
  Delay1/1 -> Sum6/1
  "if we went through a \"step\""/1 -> Hold this value/Action
  Hold this value/1(Out1) -> divide by delta T/1
  Sum6/1 -> "if we went through a \"step\""/1, Hold this value/1(In1)
  y(t)/1 -> Sum6/2, Delay1/2, Delay1/1

== system CLVF/Grab PhaseSpace Data via UDP/Use Hardware to Obtain States/Using RED, BLACK, BLUE, or RED + ARM/x_dot -> x6 ==
  note: dy/dt ~= (y2-y1)/deltaT
  y(t) : Inport
  Delay1 : Delay  DelayLength=1  InitialConditionSource=Input port
      settings: InputPortMap=u0,p4
  Hold this value : Subsystem  TreatAsAtomicUnit=on
  Sum6 : Sum  Inputs=-+|
  divide by delta T : Gain  Gain=1/serverRate
  "if we went through a \"step\"" : If  IfExpression=u1 ~= 0  ShowElse=off
  dy(t)/dt : Outport  VectorParamsAs1DForOutWhenUnconnected=off
  wires:
  divide by delta T/1 -> dy(t)/dt/1
  Delay1/1 -> Sum6/1
  "if we went through a \"step\""/1 -> Hold this value/Action
  Hold this value/1(Out1) -> divide by delta T/1
  Sum6/1 -> "if we went through a \"step\""/1, Hold this value/1(In1)
  y(t)/1 -> Sum6/2, Delay1/2, Delay1/1

== system CLVF/Grab PhaseSpace Data via UDP/Use Hardware to Obtain States/Using RED, BLACK, BLUE, or RED + ARM/x_dot -> x7 ==
  note: dy/dt ~= (y2-y1)/deltaT
  y(t) : Inport
  Delay1 : Delay  DelayLength=1  InitialConditionSource=Input port
      settings: InputPortMap=u0,p4
  Hold this value : Subsystem  TreatAsAtomicUnit=on
  Sum6 : Sum  Inputs=-+|
  divide by delta T : Gain  Gain=1/serverRate
  "if we went through a \"step\"" : If  IfExpression=u1 ~= 0  ShowElse=off
  dy(t)/dt : Outport  VectorParamsAs1DForOutWhenUnconnected=off
  wires:
  divide by delta T/1 -> dy(t)/dt/1
  Delay1/1 -> Sum6/1
  "if we went through a \"step\""/1 -> Hold this value/Action
  Hold this value/1(Out1) -> divide by delta T/1
  Sum6/1 -> "if we went through a \"step\""/1, Hold this value/1(In1)
  y(t)/1 -> Sum6/2, Delay1/2, Delay1/1

== system CLVF/Grab PhaseSpace Data via UDP/Use Hardware to Obtain States/Using RED, BLACK, BLUE, or RED + ARM/x_dot -> x8 ==
  note: dy/dt ~= (y2-y1)/deltaT
  y(t) : Inport
  Delay1 : Delay  DelayLength=1  InitialConditionSource=Input port
      settings: InputPortMap=u0,p4
  Hold this value : Subsystem  TreatAsAtomicUnit=on
  Sum6 : Sum  Inputs=-+|
  divide by delta T : Gain  Gain=1/serverRate
  "if we went through a \"step\"" : If  IfExpression=u1 ~= 0  ShowElse=off
  dy(t)/dt : Outport  VectorParamsAs1DForOutWhenUnconnected=off
  wires:
  divide by delta T/1 -> dy(t)/dt/1
  Delay1/1 -> Sum6/1
  "if we went through a \"step\""/1 -> Hold this value/Action
  Hold this value/1(Out1) -> divide by delta T/1
  Sum6/1 -> "if we went through a \"step\""/1, Hold this value/1(In1)
  y(t)/1 -> Sum6/2, Delay1/2, Delay1/1

== system CLVF/Grab PhaseSpace Data via UDP/Use Hardware to Obtain States/Using RED, BLACK, BLUE, or RED + ARM/x_dot -> x9 ==
  note: dy/dt ~= (y2-y1)/deltaT
  y(t) : Inport
  Delay1 : Delay  DelayLength=1  InitialConditionSource=Input port
      settings: InputPortMap=u0,p4
  Hold this value : Subsystem  TreatAsAtomicUnit=on
  Sum6 : Sum  Inputs=-+|
  divide by delta T : Gain  Gain=1/serverRate
  "if we went through a \"step\"" : If  IfExpression=u1 ~= 0  ShowElse=off
  dy(t)/dt : Outport  VectorParamsAs1DForOutWhenUnconnected=off
  wires:
  divide by delta T/1 -> dy(t)/dt/1
  Delay1/1 -> Sum6/1
  "if we went through a \"step\""/1 -> Hold this value/Action
  Hold this value/1(Out1) -> divide by delta T/1
  Sum6/1 -> "if we went through a \"step\""/1, Hold this value/1(In1)
  y(t)/1 -> Sum6/2, Delay1/2, Delay1/1

== system CLVF/Gyroscope & Acceleration Algorithms/Change BLACK Behavior/Fix Initial Bias/Correct GyroX ==
  In1 : Inport
  Calculate Running Mean : Subsystem  TreatAsAtomicUnit=on
  If : If  IfExpression=u1 < 5
  Pass Current Gyro : Subsystem  TreatAsAtomicUnit=on
  Subsystem : Subsystem
  Subtract : Sum  Inputs=+-
  Out1 : Outport
  wires:
  Subtract/1 -> Out1/1
  Subsystem/1(Time) -> If/1
  If/2 -> Pass Current Gyro/Action
  In1/1 -> Calculate Running Mean/1(In1), Pass Current Gyro/1(In1)
  If/1 -> Calculate Running Mean/Action
  Pass Current Gyro/1(Out1) -> Subtract/1
  Calculate Running Mean/1(Out1) -> Subtract/2

== system CLVF/Gyroscope & Acceleration Algorithms/Change BLACK Behavior/Fix Initial Bias/Correct GyroY ==
  In1 : Inport
  Calculate Running Mean : Subsystem  TreatAsAtomicUnit=on
  If : If  IfExpression=u1 < 5
  Pass Current Gyro : Subsystem  TreatAsAtomicUnit=on
  Subsystem : Subsystem
  Subtract : Sum  Inputs=+-
  Out1 : Outport
  wires:
  Subtract/1 -> Out1/1
  Subsystem/1(Time) -> If/1
  If/2 -> Pass Current Gyro/Action
  In1/1 -> Calculate Running Mean/1(In1), Pass Current Gyro/1(In1)
  If/1 -> Calculate Running Mean/Action
  Pass Current Gyro/1(Out1) -> Subtract/1
  Calculate Running Mean/1(Out1) -> Subtract/2

== system CLVF/Gyroscope & Acceleration Algorithms/Change BLACK Behavior/Fix Initial Bias/Correct GyroZ ==
  In1 : Inport
  Calculate Running Mean : Subsystem  TreatAsAtomicUnit=on
  Compare To Zero1 : simulink/Logic and Bit Operations/Compare To Zero  relop===  OutDataTypeStr=boolean
  Data Store Read1 : DataStoreRead  DataStoreName=BLACK_Rz
  Data Store Read3 : DataStoreRead  DataStoreName=BLACK_IMU_R
  Discrete-Time Integrator1 : DiscreteIntegrator  IntegratorMethod=Integration: Backward Euler  ExternalReset=either  InitialConditionSource=external  SampleTime=-1  ICPrevOutput=DiscIntNeverNeededParam  ICPrevScaledInput=DiscIntNeverNeededParam
  If : If  IfExpression=u1 < 5
  Pass Current Gyro : Subsystem  TreatAsAtomicUnit=on
  RED_Px4 : DataStoreWrite  DataStoreName=BLACK_IMU_Psi
  Subsystem : Subsystem
  Subtract : Sum  Inputs=+-
  Out1 : Outport
  wires:
  Subtract/1 -> Out1/1
  Subsystem/1(Time) -> If/1
  If/2 -> Pass Current Gyro/Action
  In1/1 -> Calculate Running Mean/1(In1), Pass Current Gyro/1(In1)
  If/1 -> Calculate Running Mean/Action
  Calculate Running Mean/1(Out1) -> Subtract/2
  Discrete-Time Integrator1/1 -> RED_Px4/1
  Compare To Zero1/1 -> Discrete-Time Integrator1/2
  Pass Current Gyro/1(Out1) -> Compare To Zero1/1, Subtract/1
  Data Store Read3/1 -> Discrete-Time Integrator1/1
  Data Store Read1/1 -> Discrete-Time Integrator1/3

== system CLVF/Gyroscope & Acceleration Algorithms/Change BLACK Behavior/Fix Initial Bias (Accel)/Correct AccelX ==
  In1 : Inport
  Calculate Running Mean : Subsystem  TreatAsAtomicUnit=on
  If : If  IfExpression=u1 < 5
  Pass Current Accel : Subsystem  TreatAsAtomicUnit=on
  Subsystem : Subsystem
  Subtract : Sum  Inputs=+-
  Out1 : Outport
  wires:
  Subtract/1 -> Out1/1
  Subsystem/1(Time) -> If/1
  If/2 -> Pass Current Accel/Action
  In1/1 -> Calculate Running Mean/1(In1), Pass Current Accel/1(In1)
  If/1 -> Calculate Running Mean/Action
  Pass Current Accel/1(Out1) -> Subtract/1
  Calculate Running Mean/1(Out1) -> Subtract/2

== system CLVF/Gyroscope & Acceleration Algorithms/Change BLACK Behavior/Fix Initial Bias (Accel)/Correct AccelY ==
  In1 : Inport
  Calculate Running Mean : Subsystem  TreatAsAtomicUnit=on
  If : If  IfExpression=u1 < 5
  Pass Current Accel : Subsystem  TreatAsAtomicUnit=on
  Subsystem : Subsystem
  Subtract : Sum  Inputs=+-
  Out1 : Outport
  wires:
  Subtract/1 -> Out1/1
  Subsystem/1(Time) -> If/1
  If/2 -> Pass Current Accel/Action
  In1/1 -> Calculate Running Mean/1(In1), Pass Current Accel/1(In1)
  If/1 -> Calculate Running Mean/Action
  Pass Current Accel/1(Out1) -> Subtract/1
  Calculate Running Mean/1(Out1) -> Subtract/2

== system CLVF/Gyroscope & Acceleration Algorithms/Change BLACK Behavior/Fix Initial Bias (Accel)/Correct AccelZ ==
  In1 : Inport
  Calculate Running Mean : Subsystem  TreatAsAtomicUnit=on
  If : If  IfExpression=u1 < 5
  Pass Current Accel : Subsystem  TreatAsAtomicUnit=on
  Subsystem : Subsystem
  Subtract : Sum  Inputs=+-
  Out1 : Outport
  wires:
  Subtract/1 -> Out1/1
  Subsystem/1(Time) -> If/1
  If/2 -> Pass Current Accel/Action
  In1/1 -> Calculate Running Mean/1(In1), Pass Current Accel/1(In1)
  If/1 -> Calculate Running Mean/Action
  Pass Current Accel/1(Out1) -> Subtract/1
  Calculate Running Mean/1(Out1) -> Subtract/2

== system CLVF/Gyroscope & Acceleration Algorithms/Change BLUE Behavior/Fix Initial Bias/Correct GyroX ==
  In1 : Inport
  Calculate Running Mean : Subsystem  TreatAsAtomicUnit=on
  If : If  IfExpression=u1 < 5
  Pass Current Gyro : Subsystem  TreatAsAtomicUnit=on
  Subsystem : Subsystem
  Subtract : Sum  Inputs=+-
  Out1 : Outport
  wires:
  Subtract/1 -> Out1/1
  Subsystem/1(Time) -> If/1
  If/2 -> Pass Current Gyro/Action
  In1/1 -> Calculate Running Mean/1(In1), Pass Current Gyro/1(In1)
  If/1 -> Calculate Running Mean/Action
  Pass Current Gyro/1(Out1) -> Subtract/1
  Calculate Running Mean/1(Out1) -> Subtract/2

== system CLVF/Gyroscope & Acceleration Algorithms/Change BLUE Behavior/Fix Initial Bias/Correct GyroY ==
  In1 : Inport
  Calculate Running Mean : Subsystem  TreatAsAtomicUnit=on
  If : If  IfExpression=u1 < 5
  Pass Current Gyro : Subsystem  TreatAsAtomicUnit=on
  Subsystem : Subsystem
  Subtract : Sum  Inputs=+-
  Out1 : Outport
  wires:
  Subtract/1 -> Out1/1
  Subsystem/1(Time) -> If/1
  If/2 -> Pass Current Gyro/Action
  In1/1 -> Calculate Running Mean/1(In1), Pass Current Gyro/1(In1)
  If/1 -> Calculate Running Mean/Action
  Pass Current Gyro/1(Out1) -> Subtract/1
  Calculate Running Mean/1(Out1) -> Subtract/2
